simulink model "BMS4Cell_Emulator"  (R2026a)
settings: Solver=daessc  StopTime=P.StopTime  MaxStep=10  RelTol=1e-4
InitFcn:
  | addpath(fullfile(fileparts(get_param(bdroot, 'FileName')), '..', 'src')); if ~exist('P','var') || ~exist('C','var'), [P, C] = params_4cell('emulator'); end
undefined symbols (not defined in the file): C, P
libraries: fl_lib x33, nesl_utility x19, ee_lib x4
settings Model: Creator=highdreameater  LastModifiedBy=highdreameater
settings DebuggingCC: AlgebraicLoopMsg=error

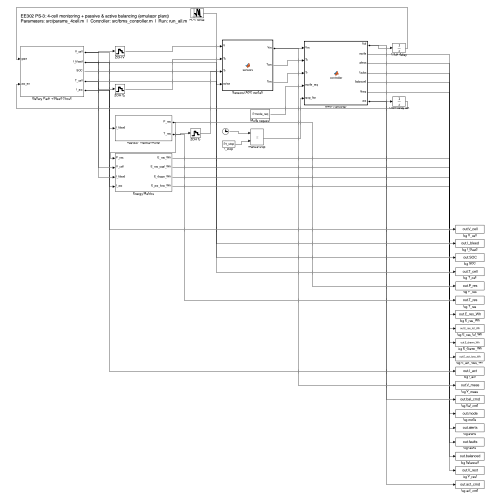
[thumbnail: Simulink's stored preview of the top-level diagram]
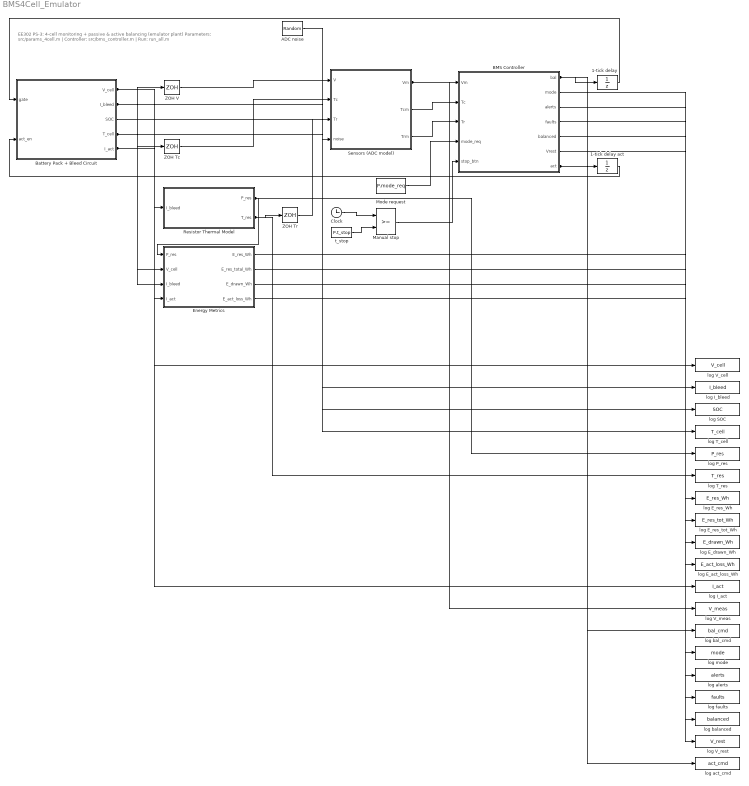
== system BMS4Cell_Emulator ==
  note: EE302 PS-3: 4-cell monitoring + passive & active balancing (emulator plant)
      | Parameters: src/params_4cell.m  |  Controller: src/bms_controller.m  |  Run: run_all.m
  1-tick delay : UnitDelay  InitialCondition=zeros(4,1)  SampleTime=C.Ts
  1-tick delay act : UnitDelay  InitialCondition=zeros(3,1)  SampleTime=C.Ts
  ADC noise : RandomNumber  Mean=zeros(4,1)  Variance=P.noise_V^2*ones(4,1)  Seed=P.seed  SampleTime=C.Ts
  BMS Controller : MATLAB Function  TreatAsAtomicUnit=on
  Battery Pack + Bleed Circuit : Subsystem
  Clock : Clock
  Energy Metrics : Subsystem
  Manual stop : RelationalOperator  OutDataTypeStr=boolean  RndMeth=Simplest  InputSameDT=off
  Mode request : Constant  Value=P.mode_req
  Resistor Thermal Model : Subsystem
  Sensors (ADC model) : MATLAB Function  TreatAsAtomicUnit=on
  ZOH Tc : ZeroOrderHold  SampleTime=C.Ts
  ZOH Tr : ZeroOrderHold  SampleTime=C.Ts
  ZOH V : ZeroOrderHold  SampleTime=C.Ts
  log E_act_loss_Wh : ToWorkspace  VariableName=E_act_loss_Wh  SaveFormat=Timeseries  SampleTime=P.log_dt
  log E_drawn_Wh : ToWorkspace  VariableName=E_drawn_Wh  SaveFormat=Timeseries  SampleTime=P.log_dt
  log E_res_Wh : ToWorkspace  VariableName=E_res_Wh  SaveFormat=Timeseries  SampleTime=P.log_dt
  log E_res_tot_Wh : ToWorkspace  VariableName=E_res_tot_Wh  SaveFormat=Timeseries  SampleTime=P.log_dt
  log I_act : ToWorkspace  VariableName=I_act  SaveFormat=Timeseries  SampleTime=P.log_dt
  log I_bleed : ToWorkspace  VariableName=I_bleed  SaveFormat=Timeseries  SampleTime=P.log_dt
  log P_res : ToWorkspace  VariableName=P_res  SaveFormat=Timeseries  SampleTime=P.log_dt
  log SOC : ToWorkspace  VariableName=SOC  SaveFormat=Timeseries  SampleTime=P.log_dt
  log T_cell : ToWorkspace  VariableName=T_cell  SaveFormat=Timeseries  SampleTime=P.log_dt
  log T_res : ToWorkspace  VariableName=T_res  SaveFormat=Timeseries  SampleTime=P.log_dt
  log V_cell : ToWorkspace  VariableName=V_cell  SaveFormat=Timeseries  SampleTime=P.log_dt
  log V_meas : ToWorkspace  VariableName=V_meas  SaveFormat=Timeseries  SampleTime=C.Ts
  log V_rest : ToWorkspace  VariableName=V_rest  SaveFormat=Timeseries  SampleTime=C.Ts
  log act_cmd : ToWorkspace  VariableName=act_cmd  SaveFormat=Timeseries  SampleTime=C.Ts
  log alerts : ToWorkspace  VariableName=alerts  SaveFormat=Timeseries  SampleTime=C.Ts
  log bal_cmd : ToWorkspace  VariableName=bal_cmd  SaveFormat=Timeseries  SampleTime=C.Ts
  log balanced : ToWorkspace  VariableName=balanced  SaveFormat=Timeseries  SampleTime=C.Ts
  log faults : ToWorkspace  VariableName=faults  SaveFormat=Timeseries  SampleTime=C.Ts
  log mode : ToWorkspace  VariableName=mode  SaveFormat=Timeseries  SampleTime=C.Ts
  t_stop : Constant  Value=P.t_stop
  wires:
  Battery Pack + Bleed Circuit/1(V_cell) -> ZOH V/1, Energy Metrics/2(V_cell), log V_cell/1
  Battery Pack + Bleed Circuit/4(T_cell) -> ZOH Tc/1, log T_cell/1
  Battery Pack + Bleed Circuit/2(I_bleed) -> Resistor Thermal Model/1(I_bleed), Energy Metrics/3(I_bleed), log I_bleed/1
  Resistor Thermal Model/2(T_res) -> ZOH Tr/1, log T_res/1
  Resistor Thermal Model/1(P_res) -> Energy Metrics/1(P_res), log P_res/1
  ZOH V/1 -> Sensors (ADC model)/1(V)
  ZOH Tc/1 -> Sensors (ADC model)/2(Tc)
  ZOH Tr/1 -> Sensors (ADC model)/3(Tr)
  ADC noise/1 -> Sensors (ADC model)/4(noise)
  Sensors (ADC model)/1(Vm) -> BMS Controller/1(Vm), log V_meas/1
  Sensors (ADC model)/2(Tcm) -> BMS Controller/2(Tc)
  Sensors (ADC model)/3(Trm) -> BMS Controller/3(Tr)
  Mode request/1 -> BMS Controller/4(mode_req)
  Clock/1 -> Manual stop/1
  t_stop/1 -> Manual stop/2
  Manual stop/1 -> BMS Controller/5(stop_btn)
  BMS Controller/1(bal) -> 1-tick delay/1, log bal_cmd/1
  1-tick delay/1 -> Battery Pack + Bleed Circuit/1(gate)
  BMS Controller/7(act) -> 1-tick delay act/1, log act_cmd/1
  1-tick delay act/1 -> Battery Pack + Bleed Circuit/2(act_en)
  Battery Pack + Bleed Circuit/5(I_act) -> Energy Metrics/4(I_act), log I_act/1
  Battery Pack + Bleed Circuit/3(SOC) -> log SOC/1
  Energy Metrics/1(E_res_Wh) -> log E_res_Wh/1
  Energy Metrics/2(E_res_total_Wh) -> log E_res_tot_Wh/1
  Energy Metrics/3(E_drawn_Wh) -> log E_drawn_Wh/1
  Energy Metrics/4(E_act_loss_Wh) -> log E_act_loss_Wh/1
  BMS Controller/2(mode) -> log mode/1
  BMS Controller/3(alerts) -> log alerts/1
  BMS Controller/4(faults) -> log faults/1
  BMS Controller/5(balanced) -> log balanced/1
  BMS Controller/6(Vrest) -> log V_rest/1

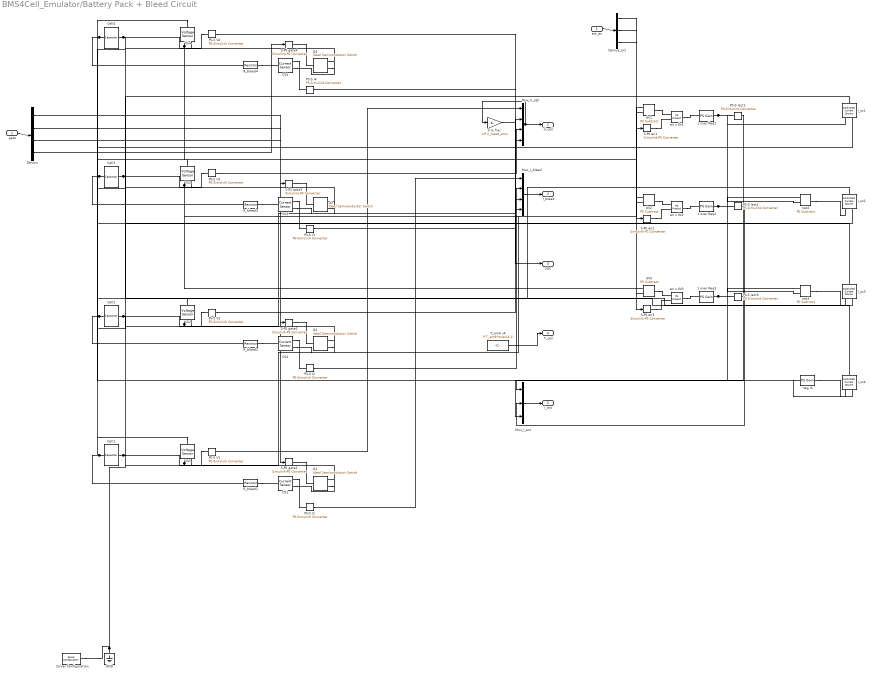
== system BMS4Cell_Emulator/Battery Pack + Bleed Circuit ==
  gate : Inport
  act_en : Inport  Port=2
  1 over Req1 : fl_lib/Physical Signals/Functions/PS Gain  gain=1/P.R_eq 1/Ohm
  1 over Req2 : fl_lib/Physical Signals/Functions/PS Gain  gain=1/P.R_eq 1/Ohm
  1 over Req3 : fl_lib/Physical Signals/Functions/PS Gain  gain=1/P.R_eq 1/Ohm
  CS{1..4} (4 alike) : fl_lib/Electrical/Electrical Sensors/Current Sensor
  Cell1 : fl_lib/Electrical/Electrical Elements/Capacitor  c=P.C_emu F  r=P.ESR_emu Ohm  g=0 1/Ohm  i_specify=off  i_priority=None  i=0 A  i_nominal_specify=off  i_nominal_value=1  i_nominal_unit=A  v_specify=off  v_priority=None  v=0 V  v_nominal_specify=off  v_nominal_value=1  v_nominal_unit=V  vc_specify=on  vc_priority=High  vc=P.Vc0_emu(1) V  vc_nominal_specify=off  vc_nominal_value=1  vc_nominal_unit=V
  Cell2 : fl_lib/Electrical/Electrical Elements/Capacitor  c=P.C_emu F  r=P.ESR_emu Ohm  g=0 1/Ohm  i_specify=off  i_priority=None  i=0 A  i_nominal_specify=off  i_nominal_value=1  i_nominal_unit=A  v_specify=off  v_priority=None  v=0 V  v_nominal_specify=off  v_nominal_value=1  v_nominal_unit=V  vc_specify=on  vc_priority=High  vc=P.Vc0_emu(2) V  vc_nominal_specify=off  vc_nominal_value=1  vc_nominal_unit=V
  Cell3 : fl_lib/Electrical/Electrical Elements/Capacitor  c=P.C_emu F  r=P.ESR_emu Ohm  g=0 1/Ohm  i_specify=off  i_priority=None  i=0 A  i_nominal_specify=off  i_nominal_value=1  i_nominal_unit=A  v_specify=off  v_priority=None  v=0 V  v_nominal_specify=off  v_nominal_value=1  v_nominal_unit=V  vc_specify=on  vc_priority=High  vc=P.Vc0_emu(3) V  vc_nominal_specify=off  vc_nominal_value=1  vc_nominal_unit=V
  Cell4 : fl_lib/Electrical/Electrical Elements/Capacitor  c=P.C_emu F  r=P.ESR_emu Ohm  g=0 1/Ohm  i_specify=off  i_priority=None  i=0 A  i_nominal_specify=off  i_nominal_value=1  i_nominal_unit=A  v_specify=off  v_priority=None  v=0 V  v_nominal_specify=off  v_nominal_value=1  v_nominal_unit=V  vc_specify=on  vc_priority=High  vc=P.Vc0_emu(4) V  vc_nominal_specify=off  vc_nominal_value=1  vc_nominal_unit=V
  Demux : Demux
  Demux_act : Demux  Outputs=3
  GND : fl_lib/Electrical/Electrical Elements/Electrical Reference
  I_sc{1..4} (4 alike) : fl_lib/Electrical/Electrical Sources/Controlled Current Source
  Mux_I_act : Mux  Inputs=3
  Mux_I_bleed : Mux
  Mux_V_cell : Mux
  PS-S I{1..4} (4 alike) : nesl_utility/PS-Simulink Converter  PhysicalDomain=network_engine_domain  SubClassName=ps_output  LeftPortType=input  RightPortType=output  PseudoPeriodic=off  Frequencies=[]  VectorFormat=inherit  Unit=A  AffineConversion=off
  PS-S Iact1 : nesl_utility/PS-Simulink Converter  PhysicalDomain=network_engine_domain  SubClassName=ps_output  LeftPortType=input  RightPortType=output  PseudoPeriodic=off  Frequencies=[]  VectorFormat=inherit  Unit=A  AffineConversion=off
  PS-S Iact2 : nesl_utility/PS-Simulink Converter  PhysicalDomain=network_engine_domain  SubClassName=ps_output  LeftPortType=input  RightPortType=output  PseudoPeriodic=off  Frequencies=[]  VectorFormat=inherit  Unit=A  AffineConversion=off
  PS-S Iact3 : nesl_utility/PS-Simulink Converter  PhysicalDomain=network_engine_domain  SubClassName=ps_output  LeftPortType=input  RightPortType=output  PseudoPeriodic=off  Frequencies=[]  VectorFormat=inherit  Unit=A  AffineConversion=off
  PS-S V{1..4} (4 alike) : nesl_utility/PS-Simulink Converter  PhysicalDomain=network_engine_domain  SubClassName=ps_output  LeftPortType=input  RightPortType=output  PseudoPeriodic=off  Frequencies=[]  VectorFormat=inherit  Unit=V  AffineConversion=off
  Q{1..4} (4 alike) : ee_lib/Semiconductors & Converters/Ideal Semiconductor Switch  port_option=ee.enum.controlport.ps  Ron=P.R_on Ohm  Goff=1e-6 1/Ohm  Vth=0.5 V  diode_param=ee.enum.semiconductors.protectionDiode.external  diode_Vf=0.8 V  diode_Ron=0.001 Ohm  diode_Goff=1e-5 1/Ohm  diode_C=50e-9 F  diode_iRM=-235 A  diode_iF=300 A  diode_idot=-50 A/us  diode_trr_param=ee.enum.converters.diodetrr.trr_factor  diode_trr_factor=3  diode_trr=15 us  diode_Qrr=1500 s*uA
  R_bleed{1..4} (4 alike) : fl_lib/Electrical/Electrical Elements/Resistor  R=P.R_bleed Ohm  i_specify=off  i_priority=None  i=0 A  i_nominal_specify=off  i_nominal_value=1  i_nominal_unit=A  v_specify=off  v_priority=None  v=0 V  v_nominal_specify=off  v_nominal_value=1  v_nominal_unit=V
  S-PS en1 : nesl_utility/Simulink-PS Converter  PhysicalDomain=network_engine_domain  SubClassName=ps_input  LeftPortType=input  RightPortType=output  PseudoPeriodic=off  Frequencies=[]  NoiseDistribution=none  NoiseParameters=[]  Unit=1  AffineConversion=off  FilteringAndDerivatives=provide  SimscapeFilterOrder=1  InputFilterTimeConstant=0.001  UdotUserProvided=0
  S-PS en2 : nesl_utility/Simulink-PS Converter  PhysicalDomain=network_engine_domain  SubClassName=ps_input  LeftPortType=input  RightPortType=output  PseudoPeriodic=off  Frequencies=[]  NoiseDistribution=none  NoiseParameters=[]  Unit=1  AffineConversion=off  FilteringAndDerivatives=provide  SimscapeFilterOrder=1  InputFilterTimeConstant=0.001  UdotUserProvided=0
  S-PS en3 : nesl_utility/Simulink-PS Converter  PhysicalDomain=network_engine_domain  SubClassName=ps_input  LeftPortType=input  RightPortType=output  PseudoPeriodic=off  Frequencies=[]  NoiseDistribution=none  NoiseParameters=[]  Unit=1  AffineConversion=off  FilteringAndDerivatives=provide  SimscapeFilterOrder=1  InputFilterTimeConstant=0.001  UdotUserProvided=0
  S-PS gate{1..4} (4 alike) : nesl_utility/Simulink-PS Converter  PhysicalDomain=network_engine_domain  SubClassName=ps_input  LeftPortType=input  RightPortType=output  PseudoPeriodic=off  Frequencies=[]  NoiseDistribution=none  NoiseParameters=[]  Unit=1  AffineConversion=off  FilteringAndDerivatives=provide  SimscapeFilterOrder=1  InputFilterTimeConstant=0.001  UdotUserProvided=0
  Solver Configuration : nesl_utility/Solver Configuration  PhysicalDomain=network_engine_domain  SubClassName=solver  LeftPortType=input  RightPortType=generic  Tones=[]  Harmonics=[]  SimulateNoise=off  Profile=off  UseLocalSampling=off  EnableSwitchedLinearOptims=on  FrequencyDomain=off  UseCCode=off  RelTol=0.001  AbsTol=0.001  MinStep=1e-09  ToWorkspace=off  RevertToSquareIcSolve=off  NumHomotopyIterations=100  PhasorMode=off  PhasorModeNumHarmonics=1  ConsistencySolver=NEWTON_XTOL_AFTER_FTOL  CanonicalOrdering=CANONICAL  OptimizeIntermediates=OPTIMIZED  IndexReductionMethod=DerivativeReplacement  DoDC=off  ResidualTolerance=1e-09  ConsistencyTolSource=GLOBAL  ConsistencyAbsTol=0.001  ConsistencyRelTol=0.001  ConsistencyTolFactor=0.001  UseLocalSolver=off  LocalSolverChoice=NE_BACKWARD_EULER_ADVANCER  ResolveIndetEquations=on  FunctionEvalNumThread=1  LocalSolverSampleTime=0.001  DoFixedCost=off  MaxNonlinIter=3  MaxModeIter=2  ComputeImpulses=off  ImpulseIterations=2  LinearAlgebra=auto  LinearAlgebraNumThread=0  EquationFormulation=NE_TIME_EF  DelaysMemoryBudget=1024  AutomaticFiltering=on  FilteringTimeConstant=0.001  PartitionStorageMethod=AS_NEEDED  PartitionMemoryBudget=1024  PartitionMethod=ROBUST  MultibodyUseLocalSolver=off  MultibodyLocalSolverChoice=ODE1  MultibodyLocalSolverSampleTime=0.001
  T_amb x4 : Constant  Value=P.T_amb*ones(4,1)
  V to frac : Gain  Gain=1/P.V_rated_emu
  VS{1..4} (4 alike) : fl_lib/Electrical/Electrical Sensors/Voltage Sensor
  dV1 : fl_lib/Physical Signals/Functions/PS Subtract
  dV2 : fl_lib/Physical Signals/Functions/PS Subtract
  dV3 : fl_lib/Physical Signals/Functions/PS Subtract
  en x dV1 : fl_lib/Physical Signals/Functions/PS Product
  en x dV2 : fl_lib/Physical Signals/Functions/PS Product
  en x dV3 : fl_lib/Physical Signals/Functions/PS Product
  neg I3 : fl_lib/Physical Signals/Functions/PS Gain  gain=-1
  net2 : fl_lib/Physical Signals/Functions/PS Subtract
  net3 : fl_lib/Physical Signals/Functions/PS Subtract
  V_cell : Outport
  I_bleed : Outport  Port=2
  SOC : Outport  Port=3
  T_cell : Outport  Port=4
  I_act : Outport  Port=5
  wires:
  gate/1 -> Demux/1
  act_en/1 -> Demux_act/1
  Mux_V_cell/1 -> V_cell/1, V to frac/1
  Mux_I_bleed/1 -> I_bleed/1
  Mux_I_act/1 -> I_act/1
  PS-S V1/1 -> Mux_V_cell/1
  PS-S I1/1 -> Mux_I_bleed/1
  Demux/1 -> S-PS gate1/1
  PS-S V2/1 -> Mux_V_cell/2
  PS-S I2/1 -> Mux_I_bleed/2
  Demux/2 -> S-PS gate2/1
  PS-S V3/1 -> Mux_V_cell/3
  PS-S I3/1 -> Mux_I_bleed/3
  Demux/3 -> S-PS gate3/1
  PS-S V4/1 -> Mux_V_cell/4
  PS-S I4/1 -> Mux_I_bleed/4
  Demux/4 -> S-PS gate4/1
  Demux_act/1 -> S-PS en1/1
  PS-S Iact1/1 -> Mux_I_act/1
  Demux_act/2 -> S-PS en2/1
  PS-S Iact2/1 -> Mux_I_act/2
  Demux_act/3 -> S-PS en3/1
  PS-S Iact3/1 -> Mux_I_act/3
  V to frac/1 -> SOC/1
  T_amb x4/1 -> T_cell/1
  connections:
  GND/LConn1 -- Solver Configuration/RConn1 -- VS1/RConn2 -- Q1/RConn2 -- Cell1/RConn1 -- I_sc1/LConn1
  VS1/LConn1 -- Cell1/LConn1 -- R_bleed1/LConn1 -- VS2/RConn2 -- Q2/RConn2 -- Cell2/RConn1 -- I_sc2/LConn1 -- I_sc1/RConn2
  PS-S V1/LConn1 -- VS1/RConn1 -- dV1/LConn1
  R_bleed1/RConn1 -- CS1/LConn1
  CS1/RConn2 -- Q1/RConn1
  CS1/RConn1 -- PS-S I1/LConn1
  S-PS gate1/RConn1 -- Q1/LConn1
  VS2/LConn1 -- Cell2/LConn1 -- R_bleed2/LConn1 -- VS3/RConn2 -- Q3/RConn2 -- Cell3/RConn1 -- I_sc3/LConn1 -- I_sc2/RConn2
  PS-S V2/LConn1 -- VS2/RConn1 -- dV1/LConn2 -- dV2/LConn1
  R_bleed2/RConn1 -- CS2/LConn1
  CS2/RConn2 -- Q2/RConn1
  CS2/RConn1 -- PS-S I2/LConn1
  S-PS gate2/RConn1 -- Q2/LConn1
  VS3/LConn1 -- Cell3/LConn1 -- R_bleed3/LConn1 -- VS4/RConn2 -- Q4/RConn2 -- Cell4/RConn1 -- I_sc4/LConn1 -- I_sc3/RConn2
  PS-S V3/LConn1 -- VS3/RConn1 -- dV2/LConn2 -- dV3/LConn1
  R_bleed3/RConn1 -- CS3/LConn1
  CS3/RConn2 -- Q3/RConn1
  CS3/RConn1 -- PS-S I3/LConn1
  S-PS gate3/RConn1 -- Q3/LConn1
  VS4/LConn1 -- Cell4/LConn1 -- R_bleed4/LConn1 -- I_sc4/RConn2
  PS-S V4/LConn1 -- VS4/RConn1 -- dV3/LConn2
  R_bleed4/RConn1 -- CS4/LConn1
  CS4/RConn2 -- Q4/RConn1
  CS4/RConn1 -- PS-S I4/LConn1
  S-PS gate4/RConn1 -- Q4/LConn1
  dV1/RConn1 -- en x dV1/LConn1
  S-PS en1/RConn1 -- en x dV1/LConn2
  en x dV1/RConn1 -- 1 over Req1/LConn1
  PS-S Iact1/LConn1 -- 1 over Req1/RConn1 -- I_sc1/RConn1 -- net2/LConn2
  dV2/RConn1 -- en x dV2/LConn1
  S-PS en2/RConn1 -- en x dV2/LConn2
  en x dV2/RConn1 -- 1 over Req2/LConn1
  PS-S Iact2/LConn1 -- 1 over Req2/RConn1 -- net2/LConn1 -- net3/LConn2
  dV3/RConn1 -- en x dV3/LConn1
  S-PS en3/RConn1 -- en x dV3/LConn2
  en x dV3/RConn1 -- 1 over Req3/LConn1
  PS-S Iact3/LConn1 -- 1 over Req3/RConn1 -- net3/LConn1 -- neg I3/LConn1
  net2/RConn1 -- I_sc2/RConn1
  net3/RConn1 -- I_sc3/RConn1
  neg I3/RConn1 -- I_sc4/RConn1

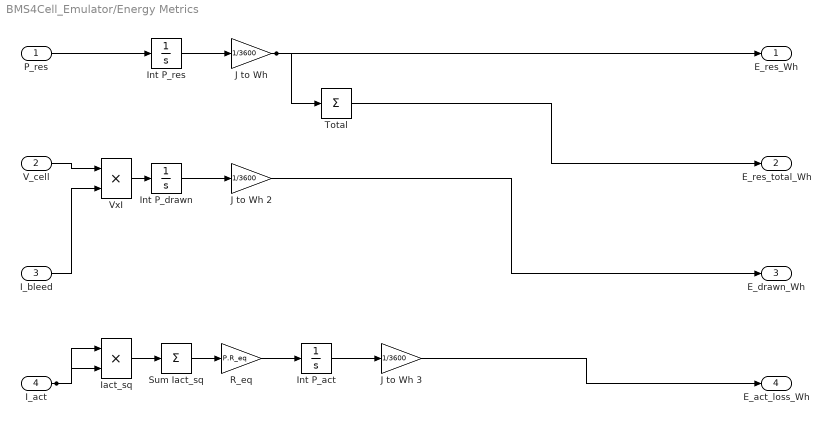
== system BMS4Cell_Emulator/Energy Metrics ==
  P_res : Inport
  V_cell : Inport  Port=2
  I_bleed : Inport  Port=3
  I_act : Inport  Port=4
  Iact_sq : Product
  Int P_act : Integrator
  Int P_drawn : Integrator
  Int P_res : Integrator
  J to Wh : Gain  Gain=1/3600
  J to Wh 2 : Gain  Gain=1/3600
  J to Wh 3 : Gain  Gain=1/3600
  R_eq : Gain  Gain=P.R_eq
  Sum Iact_sq : Sum  Inputs=+
  Total : Sum  Inputs=+
  VxI : Product
  E_res_Wh : Outport
  E_res_total_Wh : Outport  Port=2
  E_drawn_Wh : Outport  Port=3
  E_act_loss_Wh : Outport  Port=4
  wires:
  P_res/1 -> Int P_res/1
  Int P_res/1 -> J to Wh/1
  J to Wh/1 -> E_res_Wh/1, Total/1
  Total/1 -> E_res_total_Wh/1
  V_cell/1 -> VxI/1
  I_bleed/1 -> VxI/2
  VxI/1 -> Int P_drawn/1
  Int P_drawn/1 -> J to Wh 2/1
  J to Wh 2/1 -> E_drawn_Wh/1
  I_act/1 -> Iact_sq/1, Iact_sq/2
  Iact_sq/1 -> Sum Iact_sq/1
  Sum Iact_sq/1 -> R_eq/1
  R_eq/1 -> Int P_act/1
  Int P_act/1 -> J to Wh 3/1
  J to Wh 3/1 -> E_act_loss_Wh/1

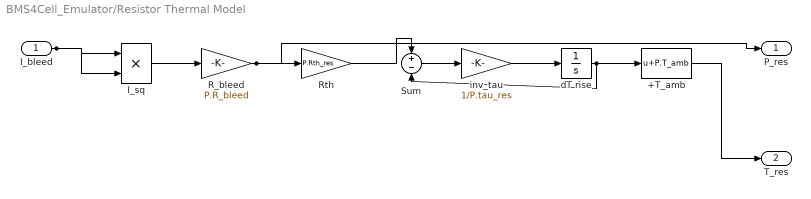
== system BMS4Cell_Emulator/Resistor Thermal Model ==
  I_bleed : Inport
  +T_amb : Bias  Bias=P.T_amb  SaturateOnIntegerOverflow=off
  I_sq : Product
  R_bleed : Gain  Gain=P.R_bleed
  Rth : Gain  Gain=P.Rth_res
  Sum : Sum  Inputs=+-
  dT rise : Integrator
  inv_tau : Gain  Gain=1/P.tau_res
  P_res : Outport
  T_res : Outport  Port=2
  wires:
  I_bleed/1 -> I_sq/1, I_sq/2
  I_sq/1 -> R_bleed/1
  R_bleed/1 -> Rth/1, P_res/1
  Rth/1 -> Sum/1
  Sum/1 -> inv_tau/1
  inv_tau/1 -> dT rise/1
  dT rise/1 -> Sum/2, +T_amb/1
  +T_amb/1 -> T_res/1

== matlab function BMS4Cell_Emulator/BMS Controller ==
  data: Vm input; bal output; Tc input; Tr input; mode_req input; stop_btn input; mode output; alerts output; faults output; balanced output; Vrest output; act output; C parameter
function [bal, mode, alerts, faults, balanced, Vrest, act] = controller(Vm, Tc, Tr, mode_req, stop_btn, C)
% Monitoring, passive/active balancing, alerts, faults, manual stop (see bms_controller.m)
[bal, mode, alerts, faults, balanced, Vrest, act] = bms_controller(Vm, Tc, Tr, mode_req, stop_btn, C);

== matlab function BMS4Cell_Emulator/Sensors (ADC model) ==
  data: V input; Vm output; Tc input; Tr input; noise input; Tcm output; Trm output; C parameter
function [Vm, Tcm, Trm] = sensors(V, Tc, Tr, noise, C)
% Measurement chain: calibration error + noise + ADC quantisation
[Vm, Tcm, Trm] = adc_measure(V, Tc, Tr, noise, C);
